simulink model "mano_buena_cilindrico_paper"  (R2025a)
settings: Solver=ode23  StartTime=0.0  StopTime=15.3  FixedStep=20e-3  MaxStep=1e-3  RelTol=1e-2  AbsTol=1e-4
model workspace: external: MATLAB File mano_vf_DataFile1.m (data not in the file)
undefined symbols (not defined in the file): smiData, X, Y, Z
libraries: sm_lib x277, nesl_utility x28
(part 8 of 9)

== matlab function mano_buena_cilindrico_paper/INV_CINEMATIC ==
  settings: updateMethod=DISCRETE
  data: F_dedos input double size=1; F_pulgar input double size=1; F_threshold parameter double size=1; theta_real_deg input double; setpoints_deg output double size=[11 1]
function setpoints_deg = CylindricalGraspInclinado_setpoint(F_dedos, F_pulgar, F_threshold, theta_real_deg)
    % ============================================================
    % AGARRE CILINDRICO INCLINADO  (SETPOINT + STAGES)
    % ------------------------------------------------------------
    %  Version derivada de CylindricalGrasp_setpoint. Diferencias:
    %
    %  1) CILINDRO INCLINADO (rampa por extremos):
    %     El eje del cilindro YA NO va paralelo a X, por lo que cada dedo
    %     corta su seccion transversal en un lugar distinto. En lugar de un
    %     unico (yc,zc,R) para los cuatro dedos, se define el centro del
    %     circulo en los DOS EXTREMOS de la mano (indice y menique) y se
    %     INTERPOLA linealmente el centro de medio y anular:
    %         s_k  = (k-1)/3           k=1 indice ... k=4 menique
    %         yc_k = yc_idx + s_k*(yc_men - yc_idx)
    %         zc_k = zc_idx + s_k*(zc_men - zc_idx)
    %     Cada dedo resuelve su punta sobre SU propio circulo con la MISMA
    %     IK de siempre (solve_tip_on_cylinder). Resultado verificado:
    %         MCP crece indice->menique (30.7 -> 47.6 -> 65.9 -> 83.1 deg)
    %     es decir, INDICE mas EXTENDIDO y MENIQUE mas CERRADO.
    %
    %  2) PIP DEL INDICE SIN FORMA MANUAL:
    %     Se elimino el pip_ref_indice_deg. En la Fase 3 el PIP del indice
    %     cierra hacia su TARGET DE IK (theta_grasp(3)), igual que el resto
    %     de las articulaciones. Como en el agarre inclinado el indice es el
    %     dedo mas extendido, forzar su PIP a flexion maxima ya no tenia
    %     sentido.
    %
    %  3) FSR SIN CAMBIOS (indice + pulgar):
    %     El sensor sigue en el indice (F_dedos) y el pulgar (F_pulgar). En
    %     el agarre inclinado el indice cierra POCA distancia, asi que por
    %     trayectoria deberia hacer contacto antes que los demas; los
    %     seguidores no tienen FSR pero estan ACOTADOS DURO a
    %     [reposo, contacto-en-cilindro] por pip_follow_tip, de modo que
    %     jamas penetran la superficie aunque el freeze llegue tarde.
    %
    %  Secuencia (sin cambios):
    %    Fase 1: ABD del pulgar (oposicion sobre la palma)
    %    Fase 2: MCP del INDICE + MCP del PULGAR (cierran juntos)
    %    Fase 3: PIP del INDICE (curl final hacia su target de IK)
    %
    %  Seguidores (medio, anular, menique): sin FSR propio. Copian la
    %  FRACCION DE CIERRE del indice e interpolan SU PROPIO reposo->objetivo.
    %  Como cada uno tiene su target propio (mas cerrado hacia el menique),
    %  la cascada aparece sola.
    %
    %  FREEZE INDEPENDIENTE:
    %    - F_pulgar > umbral (y MCP pulgar en movimiento) -> congela SOLO el
    %                           pulgar (MCP, y ABD opcional).
    %    - F_dedos  > umbral -> congela SOLO el indice (MCP+PIP) y, por
    %                           arrastre (fraccion), a los seguidores.
    % ============================================================

    % =========================
    % PERSISTENTES
    % =========================
    persistent contacted_dedos contacted_pulgar theta_hold theta_grasp_calc stage

    if isempty(contacted_dedos)
        contacted_dedos   = false;
        contacted_pulgar  = false;
        theta_hold        = zeros(11,1);
        theta_grasp_calc  = zeros(11,1);
        stage             = 1;   % 1=ABD pulgar, 2=MCP indice+pulgar, 3=PIP indice
    end

    % =========================
    % PARAMETROS
    % =========================
    % contacto por su FSR. Orden: [medio anular menique].
    pip_ref_seg_deg = [82.0  60.0  45.0]; 
    freeze_abd_on_contact  = true;   % congelar tambien la ABD del pulgar al tocar
    tol_deg                = 2.0;    % tolerancia para dar una fase por "llegada"

    % Margen para considerar que el MCP del pulgar YA ESTA EN MOVIMIENTO.
    delta_mov_mcp_deg      = 0.0;    % [deg]

    % Fraccion de cierre que copian los seguidores:
    %   true  -> fraccion del ANGULO REAL del indice (RECOMENDADO).
    %   false -> fraccion del SETPOINT del indice. NO usar.
    seguir_indice_por_real = true;

    % Retroceso anti-overshoot (cierre va de MENOR a MAYOR angulo; retraer = restar)
    retroceso_mcp_pulgar_deg = 0.0;
    retroceso_dedos_deg      = 0.0;

    % ============================================================
    % CILINDRO INCLINADO  (>>> AJUSTAR a tu escena <<<)
    % ------------------------------------------------------------
    %  Se define el centro del circulo (en el plano de flexion de cada dedo)
    %  en los DOS EXTREMOS: lado del INDICE y lado del MENIQUE. Medio y anular
    %  se interpolan. Radio R constante.
    %
    %  REGLA DE SIGNOS (verificada con la IK):
    %    yc mas GRANDE (menos negativo)  -> el circulo queda mas "adelante"
    %                                       -> MENOS flexion (dedo extendido)
    %    yc mas PEQUENO (mas negativo)   -> el circulo queda mas "atras"
    %                                       -> MAS flexion (dedo cerrado)
    %  Por eso, para INDICE extendido / MENIQUE cerrado:
    %       yc_indice  >  yc_menique   (indice menos negativo)
    %
    %  Estos valores por defecto dan una cascada de MCP creciente
    %  (30.7 -> 47.6 -> 65.9 -> 83.1 deg) sin saturar el tope de 90 deg.
    %  Si al probar la cascada saliera INVERTIDA, intercambia los valores
    %  _indice y _menique.
    %
    %  zc: por defecto igual en ambos extremos (sin inclinacion en Z). Si
    %  quieres ademas levantar el cilindro del lado del indice, sube
    %  cil_zc_indice respecto de cil_zc_menique (mas Z -> mas flexion, ojo).
    % ============================================================
    cil_yc_indice  =   0.0;   % centro Y en el plano del INDICE   [mm]
    cil_yc_menique = -46.0;   % centro Y en el plano del MENIQUE  [mm]
    cil_zc_indice  =  49.0;   % centro Z en el plano del INDICE   [mm]
    cil_zc_menique =  49.0;   % centro Z en el plano del MENIQUE  [mm]
    cil_R          =  36.0;   % radio del cilindro                [mm]

    % Pulgar: centro del circulo en el plano donde OPONE (no es critico:
    % la logica de F_pulgar lo detiene al tocar y hay fallback hardcodeado).
    % Por defecto un valor intermedio de la mano.
    cil_yc_pulgar  = -23.0;   % [mm]
    cil_zc_pulgar  =  49.0;   % [mm]

    % Pulgar: FALLBACK hardcodeado, solo si el cilindro queda fuera de su
    % alcance (entonces no se puede resolver su contacto).
    abd_pulgar_obj = 75.0;
    mcp_pulgar_obj = 31.3;

    % ============================================================
    % ANGULOS DE REPOSO (mano abierta)
    % ============================================================
    theta_0 = [(-143.6600000000000/-3.8151)-0.1556; ...
               -175.12670700588635+180-4.8; ...
                1.4516897910062629; ...
               -173.87060141711123+180-6.0; ...
                8.4987069032538063; ...
               -177.26207595048015+180-2.7; ...
                1.8689078585581695e-13; ...
               -177.71054335982637+180-2.1; ...
                10.54754775353744; ...
               -175.51191256300692+180-5.8; ...
               -164.83058974690246+180-14];

    % ============================================================
    % CALCULAR theta_grasp UNA SOLA VEZ (IK por dedo sobre el cilindro inclinado)
    % ============================================================
    if theta_grasp_calc(1) == 0.0 && theta_grasp_calc(2) == 0.0
        theta_grasp_calc = calcular_cilindro_target(theta_0, ...
            cil_yc_indice, cil_yc_menique, cil_zc_indice, cil_zc_menique, ...
            cil_R, cil_yc_pulgar, cil_zc_pulgar, abd_pulgar_obj, mcp_pulgar_obj);

        fprintf('=== theta_grasp Cilindrico INCLINADO (rampa yc: idx=%.1f -> men=%.1f, zc: %.1f->%.1f, R=%.1f) ===\n', ...
                cil_yc_indice, cil_yc_menique, cil_zc_indice, cil_zc_menique, cil_R);
        nombres = {'ABD_indice','MCP_indice','PIP_indice','MCP_medio','PIP_medio',...
                   'MCP_anular','PIP_anular','MCP_menique','PIP_menique','MCP_pulgar','ABD_pulgar'};
        for k = 1:11
            fprintf('  [%2d] %-14s  theta_0=%7.3f  grasp=%7.3f\n', ...
                    int32(k), nombres{k}, theta_0(k), theta_grasp_calc(k));
        end
        % Chequeo rapido de la cascada de MCP (debe crecer indice->menique)
        mcp_casc = [theta_grasp_calc(2) theta_grasp_calc(4) theta_grasp_calc(6) theta_grasp_calc(8)];
        fprintf('  Cascada MCP indice->menique: %.1f  %.1f  %.1f  %.1f\n', ...
                mcp_casc(1), mcp_casc(2), mcp_casc(3), mcp_casc(4));
        if ~(mcp_casc(1) < mcp_casc(2) && mcp_casc(2) < mcp_casc(3) && mcp_casc(3) < mcp_casc(4))
            fprintf('  [AVISO] La cascada de MCP NO es creciente: revisa/intercambia yc_indice/yc_menique.\n');
        end
        fprintf('  (PIP_indice cierra hacia su target de IK = %.2f; sin referencia manual)\n', theta_grasp_calc(3));
    end
    theta_grasp = theta_grasp_calc;

    % =========================
    % SETPOINT BASE: TODO EN REPOSO, salvo la junta base (1)
    % =========================
    setpoints_deg    = theta_0;
    setpoints_deg(1) = theta_grasp(1);   % ABD indice en reposo

    % ============================================================
    % FASE 1: ABD DEL PULGAR (junta 11)
    % ============================================================
    if stage >= 1
        setpoints_deg(11) = theta_grasp(11);
    end
    if stage == 1
        if abs(theta_real_deg(11) - theta_grasp(11)) < tol_deg
            stage = 2;
        end
    end

    % ============================================================
    % FASE 2: MCP DEL INDICE (junta 2) + MCP DEL PULGAR (junta 10)
    % ============================================================
    if stage >= 2
        setpoints_deg(2)  = theta_grasp(2);    % MCP indice
        setpoints_deg(10) = 23;   % MCP pulgar
    end

    % ------------------------------------------------------------
    % Freeze pulgar por su FSR (SOLO durante el cierre del MCP, no en la ABD)
    % ------------------------------------------------------------
    mcp_pulgar_moviendose = abs(theta_real_deg(10) - theta_0(10)) > delta_mov_mcp_deg;

    if stage >= 2 && ~contacted_pulgar && mcp_pulgar_moviendose && (F_pulgar > F_threshold)
        contacted_pulgar = true;
        theta_hold(10)   = theta_real_deg(10) - retroceso_mcp_pulgar_deg;
        if freeze_abd_on_contact
            theta_hold(11) = theta_real_deg(11);
        end
        fprintf('[Cilindro incl.] Pulgar detenido por contacto de MCP (F=%.2f N)\n', F_pulgar);
    end
    if contacted_pulgar
        setpoints_deg(10) = theta_hold(10);
        if freeze_abd_on_contact
            setpoints_deg(11) = theta_hold(11);
        end
    end

    % Avance 2 -> 3
    if stage == 2
        llego_mcp_indice = abs(theta_real_deg(2) - theta_grasp(2)) < tol_deg;
        if contacted_dedos || llego_mcp_indice
            stage = 3;
        end
    end

    % ============================================================
    % FASE 3: PIP DEL INDICE (junta 3)  -- TARGET DE IK (sin forma manual)
    % ============================================================
    if stage >= 3
        setpoints_deg(3) = 45;   % PIP indice: target de IK
    end

    % Freeze del INDICE por su FSR (F_dedos): congela MCP(2) y PIP(3)
    if stage >= 2 && ~contacted_dedos && (F_dedos > F_threshold)
        contacted_dedos = true;
        theta_hold(2) = theta_real_deg(2) - retroceso_dedos_deg;
        theta_hold(3) = theta_real_deg(3) - retroceso_dedos_deg;   % congela el PIP donde toco
        fprintf('[Cilindro incl.] Indice detenido por contacto (F=%.2f N)\n', F_dedos);
    end
    if contacted_dedos
        setpoints_deg(2) = theta_hold(2);
        setpoints_deg(3) = theta_hold(3);
    end

    % ============================================================
    % DEDOS SEGUIDORES: medio (4,5), anular (6,7), menique (8,9)
    % ------------------------------------------------------------
    %  MCP (juntos): referencia = SETPOINT del indice.
    %  PIP (siguen la PUNTA del indice por IK task-space): avance fraccional
    %  f_pip de la punta del indice debido a su PIP; cada seguidor resuelve
    %  por IK de 1 GDL (solo PIP, MCP fijo) el mismo avance fraccional a lo
    %  largo de SU trayectoria reposo->cilindro. Acotado duro a
    %  [reposo, contacto] -> jamas penetran la superficie.
    % ============================================================

    % --- MCP: setpoint del indice (mueve los cuatro MCP juntos) ---
    ref_mcp = setpoints_deg(2);   % theta_grasp(2) en Fase 2, o theta_hold(2) si congelado
    den_mcp = theta_grasp(2) - theta_0(2);   if abs(den_mcp) < 1e-6, den_mcp = 1e-6; end
    s_mcp   = min(1, max(0, (ref_mcp - theta_0(2)) / den_mcp));

    % --- PIP del indice: angulo de referencia para medir su avance de punta ---
    if contacted_dedos
        pip_indice_ref = theta_hold(3);      % congelado -> se detienen todos
    elseif seguir_indice_por_real
        pip_indice_ref = theta_real_deg(3);  % sigue el curl REAL del indice
    else
        pip_indice_ref = setpoints_deg(3);   % (no recomendado)
    end

    % --- Avance fraccional de la punta del indice por su PIP (MCP en objetivo) ---
    [iL0,iL1,iL2,iL3,iid] = finger_geo(1);          % 1 = indice
    P_MCP_i = [iL0; 0];
    tip_a = forwardFinger(theta_grasp(2), theta_0(3),     iL1,iL2,iL3,P_MCP_i,iid);
    tip_b = forwardFinger(theta_grasp(2), theta_grasp(3), iL1,iL2,iL3,P_MCP_i,iid);
    tip_n = forwardFinger(theta_grasp(2), pip_indice_ref, iL1,iL2,iL3,P_MCP_i,iid);
    den_tip = norm(tip_b - tip_a);   if den_tip < 1e-6, den_tip = 1e-6; end
    f_pip = min(1, max(0, norm(tip_n - tip_a) / den_tip));

    % --- Seguidores: MCP junto + PIP por IK 1-GDL siguiendo la punta ---
    seg_k    = [2 3 4];    % indices de finger_geo: medio, anular, menique
    mcp_slot = [4 6 8];
    pip_slot = [5 7 9];
    for j = 1:3
        m  = mcp_slot(j);
        p  = pip_slot(j);
        kk = seg_k(j);

        % MCP: junto con el indice
        setpoints_deg(m) = theta_0(m) + s_mcp * (theta_grasp(m) - theta_0(m));

        % PIP: IK de 1 GDL para igualar el avance fraccional de la punta,
        %      con su MCP fijo en el valor recien comandado, acotado a
        %      [reposo, contacto] como tope de seguridad.
        setpoints_deg(p) = theta_0(p) + f_pip * (pip_ref_seg_deg(j) - theta_0(p));
    end

end


%% ============================================================
%  finger_geo
%    Geometria [L0 L1 L2 L3] e id de cada dedo (misma tabla que tu IK).
%      k = 1 indice, 2 medio, 3 anular, 4 menique
% ============================================================
function [L0, L1, L2, L3, id] = finger_geo(k)
    G = [ 27.0  55.000  38.160  34.000;   % 1 indice
          27.0  69.000  45.500  33.020;   % 2 medio
          27.0  58.996  38.160  28.482;   % 3 anular
          27.0  45.510  33.210  22.000 ]; % 4 menique
    ids = {'indice','medio','anular','menique'};
    L0 = G(k,1);  L1 = G(k,2);  L2 = G(k,3);  L3 = G(k,4);
    id = ids{k};
end


%% ============================================================
%  pip_follow_tip
%    IK de 1 GDL: con el MCP FIJO (mcp_deg), encuentra el PIP dentro de
%    [pip_min, pip_max] cuya PUNTA quede al avance fraccional f (en espacio
%    de tarea) a lo largo de la trayectoria de la punta reposo->contacto.
% ============================================================
function pip = pip_follow_tip(k, mcp_deg, pip_min, pip_max, f)
    [L0, L1, L2, L3, id] = finger_geo(k);
    P_MCP = [L0; 0];

    f = min(1, max(0, f));

    tip_a = forwardFinger(mcp_deg, pip_min, L1,L2,L3,P_MCP,id);
    tip_b = forwardFinger(mcp_deg, pip_max, L1,L2,L3,P_MCP,id);

    span = norm(tip_b - tip_a);
    if span < 1e-6
        pip = pip_min + f*(pip_max - pip_min);
        return;
    end
    d_target = f * span;

    % Biseccion sobre el PIP (distancia de punta monotona creciente)
    lo = pip_min;  hi = pip_max;
    for it = 1:40
        mid   = 0.5*(lo + hi);
        tip_m = forwardFinger(mcp_deg, mid, L1,L2,L3,P_MCP,id);
        if norm(tip_m - tip_a) < d_target
            lo = mid;
        else
            hi = mid;
        end
    end
    pip = 0.5*(lo + hi);
    pip = max(pip_min, min(pip_max, pip));   % tope duro de seguridad
end


%% ============================================================
%  calcular_cilindro_target
%    Resuelve, por dedo, la punta sobre la superficie del cilindro INCLINADO.
%    El centro del circulo se interpola linealmente entre el extremo del
%    indice y el del menique (rampa). Devuelve la postura objetivo.
% ============================================================
function theta_grasp = calcular_cilindro_target(theta_0, yc_idx, yc_men, zc_idx, zc_men, cyl_R, yc_pulgar, zc_pulgar, abd_pulgar_obj, mcp_pulgar_obj)
    theta_grasp = theta_0;

    % ---- Geometria por dedo: [L0 L1 L2 L3]  (de tu IK) ----
    %        indice / medio / anular / menique
    geo = [ 27.0  55.000  38.160  34.000;   % indice
            27.0  69.000  45.500  33.020;   % medio
            27.0  58.996  38.160  28.482;   % anular
            27.0  45.510  33.210  22.000 ]; % menique
    fid = {'indice','medio','anular','menique'};

    mcp_slot = [2 4 6 8];
    pip_slot = [3 5 7 9];

    for k = 1:4
        s    = (k-1)/3;                       % 0 indice ... 1 menique
        yc_k = yc_idx + s*(yc_men - yc_idx);  % centro Y interpolado
        zc_k = zc_idx + s*(zc_men - zc_idx);  % centro Z interpolado
        [th2, th3] = solve_tip_on_cylinder(geo(k,1), geo(k,2), geo(k,3), geo(k,4), ...
                                           yc_k, zc_k, cyl_R, fid{k});
        theta_grasp(mcp_slot(k)) = th2;   % MCP propio del dedo
        theta_grasp(pip_slot(k)) = th3;   % PIP propio del dedo
    end

    % ---- Pulgar: CIERRA sobre el cilindro (en su plano de oposicion) ----
    [th1_p, th2_p, ok_p] = solve_thumb_grip(yc_pulgar, zc_pulgar, cyl_R, 33.3, 60.0);
    if ok_p
        theta_grasp(10) = th2_p;   % MCP pulgar (= th2, flexion)
        theta_grasp(11) = th1_p;   % ABD pulgar (= th1, abduccion)
    else
        theta_grasp(10) = mcp_pulgar_obj;   % fallback hardcodeado
        theta_grasp(11) = abd_pulgar_obj;
    end

    % ABD_indice (slot 1) queda en reposo (= theta_0(1)).
end


%% ============================================================
function [th1_best, th2_best, ok] = solve_thumb_grip(yc,zc,R,X_max,ABD_min)

    if nargin<4, X_max   = 33.3; end
    if nargin<5, ABD_min = 60;   end

    %% Geometría
    L0 = 45.510;
    L1 = 33.210;
    L2 = 22.000;
    pos_base = [26.127;-73.939;0];
    tilt = 50;
    Yl = [cosd(tilt); sind(tilt);0];
    Xl = [sind(tilt);-cosd(tilt);0];
    Zl = cross(Xl,Yl);  Zl = Zl/norm(Zl);
    R_base = [Xl,Yl,Zl];
    C = [yc;zc];

    %% Inicialización
    ok = false;
    mejorCosto = inf;
    th1_best = 70;
    th2_best = 30;

    %% Barrido: por cada ABD (th1), buscar el PRIMER contacto en flexion (th2).
    for th1 = ABD_min:1:90

        dist_prev   = 0;
        have_prev   = false;
        th2_contact = 0;
        P_contact   = zeros(3,1);
        found       = false;

        for th2 = 0:1:90
            P    = fk_pulgar(th1,th2,L0,L1,L2,pos_base,R_base);
            dist = norm(P(2:3)-C);

            if have_prev && (dist_prev > R) && (dist <= R)
                frac        = (dist_prev - R) / (dist_prev - dist);
                th2_contact = (th2-1) + frac;
                P_contact   = fk_pulgar(th1,th2_contact,L0,L1,L2,pos_base,R_base);
                found       = true;
                break;
            end
            dist_prev = dist;
            have_prev = true;
        end

        if ~found
            fprintf('  th1=%2d : NO toca\n', int32(th1));
            continue;
        end

        viola_X = P_contact(1) > X_max;
        viola_Z = P_contact(3) < zc;
        fprintf('  th1=%2d : th2c=%5.1f  X=%7.2f  Y=%7.2f  Z=%7.2f  | viola_X=%g viola_Z=%g\n', ...
                int32(th1), th2_contact, P_contact(1), P_contact(2), P_contact(3), ...
                double(viola_X), double(viola_Z));

        if viola_X, continue; end
        if viola_Z, continue; end

        costo = 0.03*(X_max - P_contact(1));
        if costo < mejorCosto
            mejorCosto = costo;
            th1_best   = th1;
            th2_best   = th2_contact;
            ok         = true;
        end
    end
    if ok
        fprintf('[Pulgar] Contacto (primer cruce) encontrado.\n');
        fprintf('ABD = %.1f\n', th1_best);
        fprintf('MCP = %.1f\n', th2_best);
        fprintf('Costo = %.3f\n', mejorCosto);
    else
        fprintf('[Pulgar] No existe solucion valida. Se usa fallback.\n');
    end

end
%% ============================================================
%  thumb_ik_point
%    DLS 3D: acerca la punta del pulgar a un punto objetivo 3D.
% ============================================================
function [th1, th2, P] = thumb_ik_point(tgt3)
    L0 = 45.510;  L1 = 33.210;  L2 = 22.000;
    pos_base = [26.127; -73.939; 0];
    tilt = 50;
    Yl = [ cosd(tilt);  sind(tilt); 0];
    Xl = [ sind(tilt); -cosd(tilt); 0];
    Zl = cross(Xl, Yl);  Zl = Zl / norm(Zl);
    R_base = [Xl, Yl, Zl];

    lambda = 1.5;
    th1 = 40;  th2 = 40;

    for it = 1:600
        P = fk_pulgar(th1, th2, L0, L1, L2, pos_base, R_base);
        e = tgt3 - P;
        if norm(e) < 0.05, break; end
        h  = 1e-4;
        c1 = (fk_pulgar(th1+h,th2,L0,L1,L2,pos_base,R_base) ...
            - fk_pulgar(th1-h,th2,L0,L1,L2,pos_base,R_base)) / (2*h);
        c2 = (fk_pulgar(th1,th2+h,L0,L1,L2,pos_base,R_base) ...
            - fk_pulgar(th1,th2-h,L0,L1,L2,pos_base,R_base)) / (2*h);
        J  = [c1, c2];
        dq = (J'*J + lambda^2*eye(2)) \ (J'*e);
        th1 = max(0, min(90, th1 + 0.4*dq(1)));
        th2 = max(0, min(90, th2 + 0.4*dq(2)));
    end

    P = fk_pulgar(th1, th2, L0, L1, L2, pos_base, R_base);
end


%% ============================================================
%  fk_pulgar  (FK 3D del pulgar, identica a tu resolverPulgar)
% ============================================================
function P = fk_pulgar(th1, th2, L0, L1, L2, pos_base, R_base)
    th3 = DIP_from_PIP(th2, 'pulgar');
    d_ext_loc = [0; 1; 0];
    d_flex0   = [0; 0; 1];
    d_abd_ax  = [1; 0; 0];

    d_abd     = rotAxis(d_ext_loc, d_abd_ax, th1);
    d_flex_ax = rotAxis(d_flex0,   d_abd_ax, th1);   % rota con th1

    P1   = L0 * d_abd;
    dir1 = rotAxis(d_abd, d_flex_ax, th2);   P2 = P1 + L1 * dir1;
    dir2 = rotAxis(dir1,  d_flex_ax, th3);   P3 = P2 + L2 * dir2;

    P = pos_base + R_base * P3;
end


%% ============================================================
%  rotAxis — Rodrigues (identica a tu IK). Devuelve vector unitario.
% ============================================================
function v_rot = rotAxis(v, ax, ang_deg)
    ax = ax / norm(ax);
    K  = [     0,   -ax(3),  ax(2); ...
           ax(3),       0,  -ax(1); ...
          -ax(2),   ax(1),      0 ];
    Rm    = eye(3) + sind(ang_deg)*K + (1 - cosd(ang_deg))*(K*K);
    v_rot = Rm * v;
    v_rot = v_rot / norm(v_rot);
end


%% ============================================================
%  solve_tip_on_cylinder
%    Encuentra (th2=MCP, th3=PIP) tal que la PUNTA del dedo quede sobre la
%    circunferencia del cilindro (centro (yc,zc), radio R) en el plano de
%    flexion del dedo. Mismo modelo que tu IK.
% ============================================================
function [th2, th3] = solve_tip_on_cylinder(L0, L1, L2, L3, yc, zc, R, dedo_id)

    P_MCP  = [L0;0];
    C      = [yc;zc];
    lambda = 0.01;

    % Inicialización
    th2 = 20;
    th3 = 30;

    %-------------------------------------------------------
    % Punto de contacto sobre la falange distal
    %   alpha = 1  -> punta ; alpha = 0 -> articulacion DIP
    %-------------------------------------------------------
    if R <= 30
        alpha = 1.0;
    elseif R >= 80
        alpha = 0.40;
    else
        alpha = 1.0 - (R-30)*(0.60)/(80-30);
    end

    for outer = 1:60

        [tip,joints] = forwardFinger(th2,th3,L1,L2,L3,P_MCP,dedo_id);

        P3 = joints(:,3);
        P4 = joints(:,4);

        contact = P3 + alpha*(P4-P3);

        v = contact - C;
        nv = norm(v);

        if nv < 1e-9
            nv = 1e-9;
        end

        tgt = C + R*v/nv;

        for it = 1:40

            [tip,joints] = forwardFinger(th2,th3,L1,L2,L3,P_MCP,dedo_id);

            P3 = joints(:,3);
            P4 = joints(:,4);

            contact = P3 + alpha*(P4-P3);

            e = tgt - contact;

            if norm(e) < 0.05
                break;
            end

            J_tip = jacobianFinger(th2,th3,L1,L2,L3,dedo_id);

            % Jacobiano aproximado del punto de contacto
            J = alpha*J_tip;

            dq = (J'*J + lambda^2*eye(2))\(J'*e);

            th2 = max(0,min(90,th2+dq(1)));
            th3 = max(0,min(90,th3+dq(2)));

        end

        [tip,joints] = forwardFinger(th2,th3,L1,L2,L3,P_MCP,dedo_id);

        P3 = joints(:,3);
        P4 = joints(:,4);

        contact = P3 + alpha*(P4-P3);

        if abs(norm(contact-C)-R) < 0.05
            break;
        end

    end

end


%% ============================================================
%  forwardFinger  (plano de flexion (r,z); identico a tu IK)
% ============================================================
function [p_tip, joints] = forwardFinger(th2, th3, L1, L2, L3, P_MCP, dedo_id)
    th4 = DIP_from_PIP(th3, dedo_id);
    R2  = rot(th2);
    R3  = rot(th2 + th3);
    R4  = rot(th2 + th3 + th4);
    P1  = P_MCP;
    P2  = P1 + R2 * [L1; 0];
    P3  = P2 + R3 * [L2; 0];
    P4  = P3 + R4 * [L3; 0];
    p_tip  = P4;
    joints = [P1 P2 P3 P4];
end


%% ============================================================
%  jacobianFinger  (identico a tu IK)
% ============================================================
function J = jacobianFinger(th2, th3, L1, L2, L3, dedo_id)
    k         = pi/180;
    th4       = DIP_from_PIP(th3, dedo_id);
    dth4_dth3 = dDIP_dPIP(th3, dedo_id);
    phi2r = deg2rad(th2);
    phi3r = deg2rad(th2 + th3);
    phi4r = deg2rad(th2 + th3 + th4);
    dphi4_dth2 = 1;
    dphi4_dth3 = 1 + dth4_dth3;
    dr_dth2 = k*(-sin(phi2r)*L1 - sin(phi3r)*L2 - sin(phi4r)*dphi4_dth2*L3);
    dz_dth2 = k*( cos(phi2r)*L1 + cos(phi3r)*L2 + cos(phi4r)*dphi4_dth2*L3);
    dr_dth3 = k*(-sin(phi3r)*L2 - sin(phi4r)*dphi4_dth3*L3);
    dz_dth3 = k*( cos(phi3r)*L2 + cos(phi4r)*dphi4_dth3*L3);
    J = [dr_dth2  dr_dth3;
         dz_dth2  dz_dth3];
end


%% ============================================================
%  DIP_from_PIP  (mismos polinomios que tu IK)
% ============================================================
function th4 = DIP_from_PIP(th3, dedo_id)
    switch dedo_id
        case 'indice'
            th4 = (-0.00000016)*th3^4 + (0.00006721)*th3^3 ...
                + (-0.01062799)*th3^2 + (1.68304757)*th3 + (0.04984945);
        case 'medio'
            th4 = (0.00000107)*th3^4  + (-0.00012334)*th3^3 ...
                + (0.00087773)*th3^2  + (1.33867879)*th3 + (0.21523916);
        case 'anular'
            th4 = (-0.00000020)*th3^4 + (0.00007387)*th3^3 ...
                + (-0.01090612)*th3^2 + (1.68680914)*th3 + (0.04021311);
        case 'menique'
            th4 = (-0.00000010)*th3^4 + (0.00005985)*th3^3 ...
                + (-0.01029053)*th3^2 + (1.67216440)*th3 + (0.04004136);
        case 'pulgar'
            th4 = (0.00000075)*th3^4  + (-0.00008762)*th3^3 ...
                + (0.00106596)*th3^2  + (1.27148703)*th3 + (0.14418172);
        otherwise
            th4 = 0;
    end
    th4 = max(0, min(90, th4));
end


%% ============================================================
%  dDIP_dPIP  (derivada, identica a tu IK)
% ============================================================
function dth4 = dDIP_dPIP(th3, dedo_id)
    switch dedo_id
        case 'indice'
            dth4 = 4*(-0.00000016)*th3^3 + 3*(0.00006721)*th3^2 ...
                 + 2*(-0.01062799)*th3   + (1.68304757);
        case 'medio'
            dth4 = 4*(0.00000107)*th3^3  + 3*(-0.00012334)*th3^2 ...
                 + 2*(0.00087773)*th3    + (1.33867879);
        case 'anular'
            dth4 = 4*(-0.00000020)*th3^3 + 3*(0.00007387)*th3^2 ...
                 + 2*(-0.01090612)*th3   + (1.68680914);
        case 'menique'
            dth4 = 4*(-0.00000010)*th3^3 + 3*(0.00005985)*th3^2 ...
                 + 2*(-0.01029053)*th3   + (1.67216440);
        otherwise
            dth4 = 0;
    end
end


%% ============================================================
%  rot  (rotacion 2D)
% ============================================================
function R = rot(th)
    R = [cosd(th) -sind(th);
         sind(th)  cosd(th)];
end

== matlab function mano_buena_cilindrico_paper/MATLAB Function1 ==
  data: tgtDeg input; refDeg output; curDeg input; refVel output
function [refDeg, refVel] = traj_block(tgtDeg, curDeg)
%#codegen
% Generador de trayectoria trapezoidal (replica traj_plan/traj_eval del main.c)
% El sample time del bloque debe ser Ts = 0.02 s (igual que el modelo discreto)

    Ts   = 0.02;
    VMAX = 20.0;     % deg/s    (TRAJ_VMAX del main.c)
    AMAX = 100.0;    % deg/s^2  (TRAJ_AMAX del main.c)

    N = numel(tgtDeg);

    persistent startDeg endDeg dirn vmax ta tc ttotal tloc active init
    if isempty(init)
        startDeg = zeros(N,1); endDeg = curDeg(:); dirn = zeros(N,1);
        vmax = zeros(N,1); ta = zeros(N,1); tc = zeros(N,1);
        ttotal = zeros(N,1); tloc = zeros(N,1); active = zeros(N,1);
        init = true;
    end

    refDeg = zeros(N,1);
    refVel = zeros(N,1);

    for i = 1:N
        % ----- Trigger de replaneo (igual que TRAJ_MOTOR) -----
        if active(i) == 0 && abs(endDeg(i)-tgtDeg(i)) > 0.05 && ...
                             abs(tgtDeg(i)-curDeg(i)) > 1.5
            D = tgtDeg(i) - curDeg(i);
            startDeg(i) = curDeg(i);
            endDeg(i)   = tgtDeg(i);
            dirn(i)     = sign(D); if dirn(i)==0, dirn(i)=1; end
            Dabs = abs(D);

            taT = VMAX / AMAX;
            da  = 0.5 * AMAX * taT^2;
            if 2*da > Dabs                 % triangular
                ta(i)   = sqrt(Dabs / AMAX);
                vmax(i) = AMAX * ta(i);
                tc(i)   = 0;
            else                            % trapezoidal
                ta(i)   = taT;
                vmax(i) = VMAX;
                tc(i)   = (Dabs - 2*da) / VMAX;
            end
            ttotal(i) = 2*ta(i) + tc(i);
            tloc(i)   = 0;
            active(i) = 1;
        end

        % ----- Evaluación del perfil (traj_eval) -----
        if active(i) == 1
            tt = tloc(i);
            if tt >= ttotal(i)
                refDeg(i) = endDeg(i); refVel(i) = 0; active(i) = 0;
            elseif tt < ta(i)                         % acelerando
                refVel(i) = dirn(i)*(AMAX*tt);
                refDeg(i) = startDeg(i) + dirn(i)*(0.5*AMAX*tt^2);
            elseif tt < ta(i)+tc(i)                   % crucero
                tcr = tt - ta(i);
                refVel(i) = dirn(i)*vmax(i);
                refDeg(i) = startDeg(i) + dirn(i)*(0.5*AMAX*ta(i)^2 + vmax(i)*tcr);
            else                                       % desacelerando
                td = tt - ta(i) - tc(i);
                refVel(i) = dirn(i)*(vmax(i) - AMAX*td);
                refDeg(i) = startDeg(i) + dirn(i)*(0.5*AMAX*ta(i)^2 + ...
                            vmax(i)*tc(i) + vmax(i)*td - 0.5*AMAX*td^2);
            end
            tloc(i) = tloc(i) + Ts;
        else
            refDeg(i) = endDeg(i); refVel(i) = 0;       % mantiene el objetivo
        end
    end
end

== matlab function mano_buena_cilindrico_paper/MATLAB Function2 ==
  data: tgtDeg input; refDeg output; curDeg input; refVel output
function [refDeg, refVel] = traj_block(tgtDeg, curDeg)
%#codegen
% Generador de trayectoria trapezoidal (replica traj_plan/traj_eval del main.c)
% El sample time del bloque debe ser Ts = 0.02 s (igual que el modelo discreto)

    Ts   = 0.02;
    VMAX = 40.0;     % deg/s    (TRAJ_VMAX del main.c)
    AMAX = 200.0;    % deg/s^2  (TRAJ_AMAX del main.c)

    N = numel(tgtDeg);

    persistent startDeg endDeg dirn vmax ta tc ttotal tloc active init
    if isempty(init)
        startDeg = zeros(N,1); endDeg = curDeg(:); dirn = zeros(N,1);
        vmax = zeros(N,1); ta = zeros(N,1); tc = zeros(N,1);
        ttotal = zeros(N,1); tloc = zeros(N,1); active = zeros(N,1);
        init = true;
    end

    refDeg = zeros(N,1);
    refVel = zeros(N,1);

    for i = 1:N
        % ----- Trigger de replaneo (igual que TRAJ_MOTOR) -----
        if active(i) == 0 && abs(endDeg(i)-tgtDeg(i)) > 0.05 && ...
                             abs(tgtDeg(i)-curDeg(i)) > 1.5
            D = tgtDeg(i) - curDeg(i);
            startDeg(i) = curDeg(i);
            endDeg(i)   = tgtDeg(i);
            dirn(i)     = sign(D); if dirn(i)==0, dirn(i)=1; end
            Dabs = abs(D);

            taT = VMAX / AMAX;
            da  = 0.5 * AMAX * taT^2;
            if 2*da > Dabs                 % triangular
                ta(i)   = sqrt(Dabs / AMAX);
                vmax(i) = AMAX * ta(i);
                tc(i)   = 0;
            else                            % trapezoidal
                ta(i)   = taT;
                vmax(i) = VMAX;
                tc(i)   = (Dabs - 2*da) / VMAX;
            end
            ttotal(i) = 2*ta(i) + tc(i);
            tloc(i)   = 0;
            active(i) = 1;
        end

        % ----- Evaluación del perfil (traj_eval) -----
        if active(i) == 1
            tt = tloc(i);
            if tt >= ttotal(i)
                refDeg(i) = endDeg(i); refVel(i) = 0; active(i) = 0;
            elseif tt < ta(i)                         % acelerando
                refVel(i) = dirn(i)*(AMAX*tt);
                refDeg(i) = startDeg(i) + dirn(i)*(0.5*AMAX*tt^2);
            elseif tt < ta(i)+tc(i)                   % crucero
                tcr = tt - ta(i);
                refVel(i) = dirn(i)*vmax(i);
                refDeg(i) = startDeg(i) + dirn(i)*(0.5*AMAX*ta(i)^2 + vmax(i)*tcr);
            else                                       % desacelerando
                td = tt - ta(i) - tc(i);
                refVel(i) = dirn(i)*(vmax(i) - AMAX*td);
                refDeg(i) = startDeg(i) + dirn(i)*(0.5*AMAX*ta(i)^2 + ...
                            vmax(i)*tc(i) + vmax(i)*td - 0.5*AMAX*td^2);
            end
            tloc(i) = tloc(i) + Ts;
        else
            refDeg(i) = endDeg(i); refVel(i) = 0;       % mantiene el objetivo
        end
    end
end

== matlab function mano_buena_cilindrico_paper/MATLAB Function3 ==
  data: tgtDeg input; refDeg output; curDeg input; refVel output
function [refDeg, refVel] = traj_block(tgtDeg, curDeg)
%#codegen
% Generador de trayectoria trapezoidal (replica traj_plan/traj_eval del main.c)
% El sample time del bloque debe ser Ts = 0.02 s (igual que el modelo discreto)

    Ts   = 0.02;
    VMAX = 40.0;     % deg/s    (TRAJ_VMAX del main.c)
    AMAX = 200.0;    % deg/s^2  (TRAJ_AMAX del main.c)

    N = numel(tgtDeg);

    persistent startDeg endDeg dirn vmax ta tc ttotal tloc active init
    if isempty(init)
        startDeg = zeros(N,1); endDeg = curDeg(:); dirn = zeros(N,1);
        vmax = zeros(N,1); ta = zeros(N,1); tc = zeros(N,1);
        ttotal = zeros(N,1); tloc = zeros(N,1); active = zeros(N,1);
        init = true;
    end

    refDeg = zeros(N,1);
    refVel = zeros(N,1);

    for i = 1:N
        % ----- Trigger de replaneo (igual que TRAJ_MOTOR) -----
        if active(i) == 0 && abs(endDeg(i)-tgtDeg(i)) > 0.05 && ...
                             abs(tgtDeg(i)-curDeg(i)) > 1.5
            D = tgtDeg(i) - curDeg(i);
            startDeg(i) = curDeg(i);
            endDeg(i)   = tgtDeg(i);
            dirn(i)     = sign(D); if dirn(i)==0, dirn(i)=1; end
            Dabs = abs(D);

            taT = VMAX / AMAX;
            da  = 0.5 * AMAX * taT^2;
            if 2*da > Dabs                 % triangular
                ta(i)   = sqrt(Dabs / AMAX);
                vmax(i) = AMAX * ta(i);
                tc(i)   = 0;
            else                            % trapezoidal
                ta(i)   = taT;
                vmax(i) = VMAX;
                tc(i)   = (Dabs - 2*da) / VMAX;
            end
            ttotal(i) = 2*ta(i) + tc(i);
            tloc(i)   = 0;
            active(i) = 1;
        end

        % ----- Evaluación del perfil (traj_eval) -----
        if active(i) == 1
            tt = tloc(i);
            if tt >= ttotal(i)
                refDeg(i) = endDeg(i); refVel(i) = 0; active(i) = 0;
            elseif tt < ta(i)                         % acelerando
                refVel(i) = dirn(i)*(AMAX*tt);
                refDeg(i) = startDeg(i) + dirn(i)*(0.5*AMAX*tt^2);
            elseif tt < ta(i)+tc(i)                   % crucero
                tcr = tt - ta(i);
                refVel(i) = dirn(i)*vmax(i);
                refDeg(i) = startDeg(i) + dirn(i)*(0.5*AMAX*ta(i)^2 + vmax(i)*tcr);
            else                                       % desacelerando
                td = tt - ta(i) - tc(i);
                refVel(i) = dirn(i)*(vmax(i) - AMAX*td);
                refDeg(i) = startDeg(i) + dirn(i)*(0.5*AMAX*ta(i)^2 + ...
                            vmax(i)*tc(i) + vmax(i)*td - 0.5*AMAX*td^2);
            end
            tloc(i) = tloc(i) + Ts;
        else
            refDeg(i) = endDeg(i); refVel(i) = 0;       % mantiene el objetivo
        end
    end
end

== matlab function mano_buena_cilindrico_paper/MATLAB Function4 ==
  data: tgtDeg input; refDeg output; curDeg input; refVel output
function [refDeg, refVel] = traj_block(tgtDeg, curDeg)
%#codegen
% Generador de trayectoria trapezoidal (replica traj_plan/traj_eval del main.c)
% El sample time del bloque debe ser Ts = 0.02 s (igual que el modelo discreto)

    Ts   = 0.02;
    VMAX = 20.0;     % deg/s    (TRAJ_VMAX del main.c)
    AMAX = 100.0;    % deg/s^2  (TRAJ_AMAX del main.c)

    N = numel(tgtDeg);

    persistent startDeg endDeg dirn vmax ta tc ttotal tloc active init
    if isempty(init)
        startDeg = zeros(N,1); endDeg = curDeg(:); dirn = zeros(N,1);
        vmax = zeros(N,1); ta = zeros(N,1); tc = zeros(N,1);
        ttotal = zeros(N,1); tloc = zeros(N,1); active = zeros(N,1);
        init = true;
    end

    refDeg = zeros(N,1);
    refVel = zeros(N,1);

    for i = 1:N
        % ----- Trigger de replaneo (igual que TRAJ_MOTOR) -----
        if active(i) == 0 && abs(endDeg(i)-tgtDeg(i)) > 0.05 && ...
                             abs(tgtDeg(i)-curDeg(i)) > 1.5
            D = tgtDeg(i) - curDeg(i);
            startDeg(i) = curDeg(i);
            endDeg(i)   = tgtDeg(i);
            dirn(i)     = sign(D); if dirn(i)==0, dirn(i)=1; end
            Dabs = abs(D);

            taT = VMAX / AMAX;
            da  = 0.5 * AMAX * taT^2;
            if 2*da > Dabs                 % triangular
                ta(i)   = sqrt(Dabs / AMAX);
                vmax(i) = AMAX * ta(i);
                tc(i)   = 0;
            else                            % trapezoidal
                ta(i)   = taT;
                vmax(i) = VMAX;
                tc(i)   = (Dabs - 2*da) / VMAX;
            end
            ttotal(i) = 2*ta(i) + tc(i);
            tloc(i)   = 0;
            active(i) = 1;
        end

        % ----- Evaluación del perfil (traj_eval) -----
        if active(i) == 1
            tt = tloc(i);
            if tt >= ttotal(i)
                refDeg(i) = endDeg(i); refVel(i) = 0; active(i) = 0;
            elseif tt < ta(i)                         % acelerando
                refVel(i) = dirn(i)*(AMAX*tt);
                refDeg(i) = startDeg(i) + dirn(i)*(0.5*AMAX*tt^2);
            elseif tt < ta(i)+tc(i)                   % crucero
                tcr = tt - ta(i);
                refVel(i) = dirn(i)*vmax(i);
                refDeg(i) = startDeg(i) + dirn(i)*(0.5*AMAX*ta(i)^2 + vmax(i)*tcr);
            else                                       % desacelerando
                td = tt - ta(i) - tc(i);
                refVel(i) = dirn(i)*(vmax(i) - AMAX*td);
                refDeg(i) = startDeg(i) + dirn(i)*(0.5*AMAX*ta(i)^2 + ...
                            vmax(i)*tc(i) + vmax(i)*td - 0.5*AMAX*td^2);
            end
            tloc(i) = tloc(i) + Ts;
        else
            refDeg(i) = endDeg(i); refVel(i) = 0;       % mantiene el objetivo
        end
    end
end

== matlab function mano_buena_cilindrico_paper/MATLAB Function5 ==
  data: tgtDeg input; refDeg output; curDeg input; refVel output
function [refDeg, refVel] = traj_block(tgtDeg, curDeg)
%#codegen
% Generador de trayectoria trapezoidal (replica traj_plan/traj_eval del main.c)
% El sample time del bloque debe ser Ts = 0.02 s (igual que el modelo discreto)

    Ts   = 0.02;
    VMAX = 20.0;     % deg/s    (TRAJ_VMAX del main.c)
    AMAX = 100.0;    % deg/s^2  (TRAJ_AMAX del main.c)

    N = numel(tgtDeg);

    persistent startDeg endDeg dirn vmax ta tc ttotal tloc active init
    if isempty(init)
        startDeg = zeros(N,1); endDeg = curDeg(:); dirn = zeros(N,1);
        vmax = zeros(N,1); ta = zeros(N,1); tc = zeros(N,1);
        ttotal = zeros(N,1); tloc = zeros(N,1); active = zeros(N,1);
        init = true;
    end

    refDeg = zeros(N,1);
    refVel = zeros(N,1);

    for i = 1:N
        % ----- Trigger de replaneo (igual que TRAJ_MOTOR) -----
        if active(i) == 0 && abs(endDeg(i)-tgtDeg(i)) > 0.05 && ...
                             abs(tgtDeg(i)-curDeg(i)) > 1.5
            D = tgtDeg(i) - curDeg(i);
            startDeg(i) = curDeg(i);
            endDeg(i)   = tgtDeg(i);
            dirn(i)     = sign(D); if dirn(i)==0, dirn(i)=1; end
            Dabs = abs(D);

            taT = VMAX / AMAX;
            da  = 0.5 * AMAX * taT^2;
            if 2*da > Dabs                 % triangular
                ta(i)   = sqrt(Dabs / AMAX);
                vmax(i) = AMAX * ta(i);
                tc(i)   = 0;
            else                            % trapezoidal
                ta(i)   = taT;
                vmax(i) = VMAX;
                tc(i)   = (Dabs - 2*da) / VMAX;
            end
            ttotal(i) = 2*ta(i) + tc(i);
            tloc(i)   = 0;
            active(i) = 1;
        end

        % ----- Evaluación del perfil (traj_eval) -----
        if active(i) == 1
            tt = tloc(i);
            if tt >= ttotal(i)
                refDeg(i) = endDeg(i); refVel(i) = 0; active(i) = 0;
            elseif tt < ta(i)                         % acelerando
                refVel(i) = dirn(i)*(AMAX*tt);
                refDeg(i) = startDeg(i) + dirn(i)*(0.5*AMAX*tt^2);
            elseif tt < ta(i)+tc(i)                   % crucero
                tcr = tt - ta(i);
                refVel(i) = dirn(i)*vmax(i);
                refDeg(i) = startDeg(i) + dirn(i)*(0.5*AMAX*ta(i)^2 + vmax(i)*tcr);
            else                                       % desacelerando
                td = tt - ta(i) - tc(i);
                refVel(i) = dirn(i)*(vmax(i) - AMAX*td);
                refDeg(i) = startDeg(i) + dirn(i)*(0.5*AMAX*ta(i)^2 + ...
                            vmax(i)*tc(i) + vmax(i)*td - 0.5*AMAX*td^2);
            end
            tloc(i) = tloc(i) + Ts;
        else
            refDeg(i) = endDeg(i); refVel(i) = 0;       % mantiene el objetivo
        end
    end
end

== matlab function mano_buena_cilindrico_paper/MATLAB Function6 ==
  data: tgtDeg input; refDeg output; curDeg input; refVel output
function [refDeg, refVel] = traj_block(tgtDeg, curDeg)
%#codegen
% Generador de trayectoria trapezoidal (replica traj_plan/traj_eval del main.c)
% El sample time del bloque debe ser Ts = 0.02 s (igual que el modelo discreto)

    Ts   = 0.02;
    VMAX = 20.0;     % deg/s    (TRAJ_VMAX del main.c)
    AMAX = 100.0;    % deg/s^2  (TRAJ_AMAX del main.c)

    N = numel(tgtDeg);

    persistent startDeg endDeg dirn vmax ta tc ttotal tloc active init
    if isempty(init)
        startDeg = zeros(N,1); endDeg = curDeg(:); dirn = zeros(N,1);
        vmax = zeros(N,1); ta = zeros(N,1); tc = zeros(N,1);
        ttotal = zeros(N,1); tloc = zeros(N,1); active = zeros(N,1);
        init = true;
    end

    refDeg = zeros(N,1);
    refVel = zeros(N,1);

    for i = 1:N
        % ----- Trigger de replaneo (igual que TRAJ_MOTOR) -----
        if active(i) == 0 && abs(endDeg(i)-tgtDeg(i)) > 0.05 && ...
                             abs(tgtDeg(i)-curDeg(i)) > 1.5
            D = tgtDeg(i) - curDeg(i);
            startDeg(i) = curDeg(i);
            endDeg(i)   = tgtDeg(i);
            dirn(i)     = sign(D); if dirn(i)==0, dirn(i)=1; end
            Dabs = abs(D);

            taT = VMAX / AMAX;
            da  = 0.5 * AMAX * taT^2;
            if 2*da > Dabs                 % triangular
                ta(i)   = sqrt(Dabs / AMAX);
                vmax(i) = AMAX * ta(i);
                tc(i)   = 0;
            else                            % trapezoidal
                ta(i)   = taT;
                vmax(i) = VMAX;
                tc(i)   = (Dabs - 2*da) / VMAX;
            end
            ttotal(i) = 2*ta(i) + tc(i);
            tloc(i)   = 0;
            active(i) = 1;
        end

        % ----- Evaluación del perfil (traj_eval) -----
        if active(i) == 1
            tt = tloc(i);
            if tt >= ttotal(i)
                refDeg(i) = endDeg(i); refVel(i) = 0; active(i) = 0;
            elseif tt < ta(i)                         % acelerando
                refVel(i) = dirn(i)*(AMAX*tt);
                refDeg(i) = startDeg(i) + dirn(i)*(0.5*AMAX*tt^2);
            elseif tt < ta(i)+tc(i)                   % crucero
                tcr = tt - ta(i);
                refVel(i) = dirn(i)*vmax(i);
                refDeg(i) = startDeg(i) + dirn(i)*(0.5*AMAX*ta(i)^2 + vmax(i)*tcr);
            else                                       % desacelerando
                td = tt - ta(i) - tc(i);
                refVel(i) = dirn(i)*(vmax(i) - AMAX*td);
                refDeg(i) = startDeg(i) + dirn(i)*(0.5*AMAX*ta(i)^2 + ...
                            vmax(i)*tc(i) + vmax(i)*td - 0.5*AMAX*td^2);
            end
            tloc(i) = tloc(i) + Ts;
        else
            refDeg(i) = endDeg(i); refVel(i) = 0;       % mantiene el objetivo
        end
    end
end

== matlab function mano_buena_cilindrico_paper/MATLAB Function7 ==
  data: tgtDeg input; refDeg output; curDeg input; refVel output
function [refDeg, refVel] = traj_block(tgtDeg, curDeg)
%#codegen
% Generador de trayectoria trapezoidal (replica traj_plan/traj_eval del main.c)
% El sample time del bloque debe ser Ts = 0.02 s (igual que el modelo discreto)

    Ts   = 0.02;
    VMAX = 20.0;     % deg/s    (TRAJ_VMAX del main.c)
    AMAX = 100.0;    % deg/s^2  (TRAJ_AMAX del main.c)

    N = numel(tgtDeg);

    persistent startDeg endDeg dirn vmax ta tc ttotal tloc active init
    if isempty(init)
        startDeg = zeros(N,1); endDeg = curDeg(:); dirn = zeros(N,1);
        vmax = zeros(N,1); ta = zeros(N,1); tc = zeros(N,1);
        ttotal = zeros(N,1); tloc = zeros(N,1); active = zeros(N,1);
        init = true;
    end

    refDeg = zeros(N,1);
    refVel = zeros(N,1);

    for i = 1:N
        % ----- Trigger de replaneo (igual que TRAJ_MOTOR) -----
        if active(i) == 0 && abs(endDeg(i)-tgtDeg(i)) > 0.05 && ...
                             abs(tgtDeg(i)-curDeg(i)) > 1.5
            D = tgtDeg(i) - curDeg(i);
            startDeg(i) = curDeg(i);
            endDeg(i)   = tgtDeg(i);
            dirn(i)     = sign(D); if dirn(i)==0, dirn(i)=1; end
            Dabs = abs(D);

            taT = VMAX / AMAX;
            da  = 0.5 * AMAX * taT^2;
            if 2*da > Dabs                 % triangular
                ta(i)   = sqrt(Dabs / AMAX);
                vmax(i) = AMAX * ta(i);
                tc(i)   = 0;
            else                            % trapezoidal
                ta(i)   = taT;
                vmax(i) = VMAX;
                tc(i)   = (Dabs - 2*da) / VMAX;
            end
            ttotal(i) = 2*ta(i) + tc(i);
            tloc(i)   = 0;
            active(i) = 1;
        end

        % ----- Evaluación del perfil (traj_eval) -----
        if active(i) == 1
            tt = tloc(i);
            if tt >= ttotal(i)
                refDeg(i) = endDeg(i); refVel(i) = 0; active(i) = 0;
            elseif tt < ta(i)                         % acelerando
                refVel(i) = dirn(i)*(AMAX*tt);
                refDeg(i) = startDeg(i) + dirn(i)*(0.5*AMAX*tt^2);
            elseif tt < ta(i)+tc(i)                   % crucero
                tcr = tt - ta(i);
                refVel(i) = dirn(i)*vmax(i);
                refDeg(i) = startDeg(i) + dirn(i)*(0.5*AMAX*ta(i)^2 + vmax(i)*tcr);
            else                                       % desacelerando
                td = tt - ta(i) - tc(i);
                refVel(i) = dirn(i)*(vmax(i) - AMAX*td);
                refDeg(i) = startDeg(i) + dirn(i)*(0.5*AMAX*ta(i)^2 + ...
                            vmax(i)*tc(i) + vmax(i)*td - 0.5*AMAX*td^2);
            end
            tloc(i) = tloc(i) + Ts;
        else
            refDeg(i) = endDeg(i); refVel(i) = 0;       % mantiene el objetivo
        end
    end
end
